simulink library "Multibody_Parts_Lib"  (R2024a)
settings: Solver=VariableStepAuto  StartTime=0.0  StopTime=10.0  RelTol=1e-3
undefined symbols (not defined in the file or in its folder): b_gear_pd_asy, b_radius_asy, b_visc_frict_asy, bevel_angle_asy, bevel_angle_bf_asy, bevel_angle_fg_asy, f_gear_pd_asy, f_radius_asy, f_visc_frict_asy, g_radius_asy, g_visc_frict_asy, gear_ra_asy, gear_visc_frict_asy, Hand, Left, Local, pinion_pd_asy, screw_lead, worm_lead_angle_asy, worm_rad_asy, worm_visc_frict_asy, X, Y, Z
libraries: sm_lib x143, $bdroot x22, nesl_utility x16
(part 6 of 6)

== system Multibody_Parts_Lib/Gears/Assemblies/Bevel Gear Assembly ==
  Constraints : $bdroot/Gears/Assemblies/Bevel Gear Constraints  bevel_angle=bevel_angle_asy  b_radius=b_radius_asy  f_radius=f_radius_asy  b_visc_frict=b_visc_frict_asy  f_visc_frict=f_visc_frict_asy
  Gear B : $bdroot/Gears/Bevel Gear  gear_ra=b_radius_asy  gear_th=b_thickness_asy  gear_ca=b_cone_angle_asy  gear_hr=b_hole_radius_asy  gear_rho=b_rho_asy  gear_clr=b_clr_asy  gear_opc=b_opc_asy  popup_markings=Two  mark_radius_range=b_mark_radius_range  mark_angle_range=b_mark_angle_range  mark_color=b_mark_clr
  Gear F : $bdroot/Gears/Bevel Gear  gear_ra=f_radius_asy  gear_th=f_thickness_asy  gear_ca=bevel_angle_asy-b_cone_angle_asy  gear_hr=f_hole_radius_asy  gear_rho=f_rho_asy  gear_clr=f_clr_asy  gear_opc=f_opc_asy  popup_markings=Two  mark_radius_range=f_mark_radius_range  mark_angle_range=f_mark_angle_range  mark_color=f_mark_clr
  F : PMIOPort  Side=Left
  B : PMIOPort  Port=2  Side=Left
  H : PMIOPort  Port=3  Side=Left
  connections:
  Constraints/LConn2 -- Gear B/RConn1 -- B/RConn1
  Constraints/LConn1 -- Gear F/RConn1 -- F/RConn1
  Constraints/LConn3 -- H/RConn1

== system Multibody_Parts_Lib/Gears/Assemblies/Common Gear Constraints ==
  Common Gear Constraint : sm_lib/Gears and Couplings/Gears/Common Gear Constraint  GearType=External  SpecificationType=PitchCircleRadii  CenterDistance=30  CenterDistanceUnits=cm  GearRatio=0.5  BaseGearRadius=b_gear_pd/2  BaseGearRadiusUnits=m  FollGearRadius=f_gear_pd/2  FollGearRadiusUnits=m
  Revolute Gear B : sm_lib/Joints/Revolute Joint  JointMode=Normal  CompositeWrenchDir=FollowerOnBase  CompositeWrenchFrame=BaseFrame  SenseConstraintForce=off  SenseConstraintTorque=off  SenseTotalForce=off  SenseTotalTorque=off  PositionTargetSpecify=off  PositionTargetPriority=High  PositionTargetValue=0  PositionTargetValueUnits=deg  VelocityTargetSpecify=off  VelocityTargetPriority=High  VelocityTargetValue=0  VelocityTargetValueUnits=deg/s  EquilibriumPosition=0  EquilibriumPositionUnits=deg  SpringStiffness=0  SpringStiffnessUnits=N*m/deg  DampingCoefficient=b_visc_frict  DampingCoefficientUnits=N*m/(deg/s)  LowerLimitSpecify=off  LowerLimitBound=-90  LowerLimitBoundUnits=deg  LowerLimitStiffness=1e4  LowerLimitStiffnessUnits=N*m/deg  LowerLimitDamping=10  LowerLimitDampingUnits=N*m/(deg/s)  LowerLimitTransitionRegionWidth=0.1  LowerLimitTransitionRegionWidthUnits=deg  UpperLimitSpecify=off  UpperLimitBound=90  UpperLimitBoundUnits=deg  UpperLimitStiffness=1e4  UpperLimitStiffnessUnits=N*m/deg  UpperLimitDamping=10  UpperLimitDampingUnits=N*m/(deg/s)  UpperLimitTransitionRegionWidth=0.1  UpperLimitTransitionRegionWidthUnits=deg  TorqueActuationMode=NoTorque  MotionActuationMode=ComputedMotion  SensePosition=off  SenseVelocity=off  SenseAcceleration=off  SenseTorqueForce=off  SenseLowerLimitTorqueForce=off  SenseUpperLimitTorqueForce=off
  Revolute Gear F : sm_lib/Joints/Revolute Joint  JointMode=Normal  CompositeWrenchDir=FollowerOnBase  CompositeWrenchFrame=BaseFrame  SenseConstraintForce=off  SenseConstraintTorque=off  SenseTotalForce=off  SenseTotalTorque=off  PositionTargetSpecify=on  PositionTargetPriority=High  PositionTargetValue=45  PositionTargetValueUnits=deg  VelocityTargetSpecify=off  VelocityTargetPriority=High  VelocityTargetValue=0  VelocityTargetValueUnits=deg/s  EquilibriumPosition=0  EquilibriumPositionUnits=deg  SpringStiffness=0  SpringStiffnessUnits=N*m/deg  DampingCoefficient=f_visc_frict  DampingCoefficientUnits=N*m/(deg/s)  LowerLimitSpecify=off  LowerLimitBound=-90  LowerLimitBoundUnits=deg  LowerLimitStiffness=1e4  LowerLimitStiffnessUnits=N*m/deg  LowerLimitDamping=10  LowerLimitDampingUnits=N*m/(deg/s)  LowerLimitTransitionRegionWidth=0.1  LowerLimitTransitionRegionWidthUnits=deg  UpperLimitSpecify=off  UpperLimitBound=90  UpperLimitBoundUnits=deg  UpperLimitStiffness=1e4  UpperLimitStiffnessUnits=N*m/deg  UpperLimitDamping=10  UpperLimitDampingUnits=N*m/(deg/s)  UpperLimitTransitionRegionWidth=0.1  UpperLimitTransitionRegionWidthUnits=deg  TorqueActuationMode=NoTorque  MotionActuationMode=ComputedMotion  SensePosition=off  SenseVelocity=off  SenseAcceleration=off  SenseTorqueForce=off  SenseLowerLimitTorqueForce=off  SenseUpperLimitTorqueForce=off
  Transform Gear F : sm_lib/Frames and Transforms/Rigid Transform  RotationMethod=None  FollAlignAxisA=+X  BaseAlignAxisA=+Y  FollAlignAxisB=+Y  BaseAlignAxisB=+Z  RotationStandardAxis=+Z  RotationAngle=0  RotationAngleUnits=deg  RotationArbitraryAxis=[0 0 1]  RotationSequenceAxes=FollowerAxes  RotationSequence=XYX  RotationSequenceAngles=[0 0 0]  RotationSequenceAnglesUnits=deg  RotationMatrix=[1 0 0; 0 1 0; 0 0 1]  Quaternion=[1 0 0 0]  TranslationMethod=StandardAxis  TranslationCartesianOffset=[0 0 0]  TranslationCartesianOffsetUnits=m  TranslationStandardAxis=+X  TranslationStandardOffset=gear_axis_offset  TranslationStandardOffsetUnits=m  TranslationROffset=0  TranslationROffsetUnits=m  TranslationThetaOffset=0  TranslationThetaOffsetUnits=deg  TranslationZOffset=0  TranslationZOffsetUnits=m
  F : PMIOPort  Side=Left
  B : PMIOPort  Port=2  Side=Left
  H : PMIOPort  Port=3  Side=Left
  connections:
  Revolute Gear B/RConn1 -- Common Gear Constraint/LConn1 -- B/RConn1
  Revolute Gear F/RConn1 -- Common Gear Constraint/RConn1 -- F/RConn1
  Transform Gear F/RConn1 -- Revolute Gear F/LConn1
  H/RConn1 -- Transform Gear F/LConn1 -- Revolute Gear B/LConn1

== system Multibody_Parts_Lib/Gears/Assemblies/Common Gear Assembly ==
  Constraints : $bdroot/Gears/Assemblies/Common Gear Constraints  popup_gear_type=External  b_gear_pd=b_gear_pd_asy  f_gear_pd=f_gear_pd_asy  b_visc_frict=b_visc_frict_asy  f_visc_frict=f_visc_frict_asy
  Gear B : $bdroot/Gears/Gear  popup_gear_type=External  gear_pd=b_gear_pd_asy  gear_nt=b_gear_nt  gear_th=b_gear_th  gear_rh=b_gear_rh  gear_rt=pinion_rt  gear_rho=b_gear_rho  gear_clr=b_gear_clr  gear_opc=b_gear_opc  popup_ad_dd=Specify  gear_ad=b_gear_ad  gear_dd=b_gear_dd  popup_markings=Two  mark_radius_range=b_mark_radius_range  mark_angle_range=b_mark_angle_range  mark_color=b_mark_color
  Gear F : $bdroot/Gears/Gear  popup_gear_type=External  gear_pd=f_gear_pd_asy  gear_nt=f_gear_nt  gear_th=f_gear_th  gear_rh=f_gear_rht  gear_rt=f_gear_rht  gear_rho=f_gear_rho  gear_clr=f_gear_clr  gear_opc=f_gear_opc  popup_ad_dd=Specify  gear_ad=f_gear_ad  gear_dd=f_gear_dd  popup_markings=Two  mark_radius_range=f_mark_radius_range  mark_angle_range=f_mark_angle_range  mark_color=f_mark_color
  Transform B Offset Angle : sm_lib/Frames and Transforms/Rigid Transform  RotationMethod=StandardAxis  FollAlignAxisA=+X  BaseAlignAxisA=+Y  FollAlignAxisB=+Y  BaseAlignAxisB=+Z  RotationStandardAxis=+Z  RotationAngle=b_gear_offset_angle  RotationAngleUnits=deg  RotationArbitraryAxis=[0 0 1]  RotationSequenceAxes=FollowerAxes  RotationSequence=XYX  RotationSequenceAngles=[0 0 0]  RotationSequenceAnglesUnits=deg  RotationMatrix=[1 0 0; 0 1 0; 0 0 1]  Quaternion=[1 0 0 0]  TranslationMethod=None  TranslationCartesianOffset=[0 0 0]  TranslationCartesianOffsetUnits=m  TranslationStandardAxis=+Z  TranslationStandardOffset=0  TranslationStandardOffsetUnits=m  TranslationROffset=0  TranslationROffsetUnits=m  TranslationThetaOffset=0  TranslationThetaOffsetUnits=deg  TranslationZOffset=0  TranslationZOffsetUnits=m
  Transform F Offset Angle : sm_lib/Frames and Transforms/Rigid Transform  RotationMethod=StandardAxis  FollAlignAxisA=+X  BaseAlignAxisA=+Y  FollAlignAxisB=+Y  BaseAlignAxisB=+Z  RotationStandardAxis=+Z  RotationAngle=f_gear_offset_angle  RotationAngleUnits=deg  RotationArbitraryAxis=[0 0 1]  RotationSequenceAxes=FollowerAxes  RotationSequence=XYX  RotationSequenceAngles=[0 0 0]  RotationSequenceAnglesUnits=deg  RotationMatrix=[1 0 0; 0 1 0; 0 0 1]  Quaternion=[1 0 0 0]  TranslationMethod=None  TranslationCartesianOffset=[0 0 0]  TranslationCartesianOffsetUnits=m  TranslationStandardAxis=+Z  TranslationStandardOffset=0  TranslationStandardOffsetUnits=m  TranslationROffset=0  TranslationROffsetUnits=m  TranslationThetaOffset=0  TranslationThetaOffsetUnits=deg  TranslationZOffset=0  TranslationZOffsetUnits=m
  F : PMIOPort  Side=Left
  B : PMIOPort  Port=2  Side=Left
  H : PMIOPort  Port=3  Side=Left
  connections:
  Constraints/LConn3 -- H/RConn1
  Gear B/RConn1 -- Transform B Offset Angle/RConn1
  Gear F/RConn1 -- Transform F Offset Angle/RConn1
  F/RConn1 -- Constraints/LConn1 -- Transform F Offset Angle/LConn1
  Constraints/LConn2 -- B/RConn1 -- Transform B Offset Angle/LConn1

== system Multibody_Parts_Lib/Gears/Assemblies/Rack and Pinion Constraints ==
  Check Frames Rack and Pinion : Subsystem
  Prismatic Rack : sm_lib/Joints/Prismatic Joint  JointMode=Normal  CompositeWrenchDir=FollowerOnBase  CompositeWrenchFrame=BaseFrame  SenseConstraintForce=off  SenseConstraintTorque=off  SenseTotalForce=off  SenseTotalTorque=off  PositionTargetSpecify=off  PositionTargetPriority=High  PositionTargetValue=0  PositionTargetValueUnits=m  VelocityTargetSpecify=off  VelocityTargetPriority=High  VelocityTargetValue=0  VelocityTargetValueUnits=m/s  EquilibriumPosition=0  EquilibriumPositionUnits=m  SpringStiffness=0  SpringStiffnessUnits=N/m  DampingCoefficient=rack_visc_frict  DampingCoefficientUnits=N/(m/s)  LowerLimitSpecify=off  LowerLimitBound=-1  LowerLimitBoundUnits=m  LowerLimitStiffness=1e6  LowerLimitStiffnessUnits=N/m  LowerLimitDamping=1e3  LowerLimitDampingUnits=N/(m/s)  LowerLimitTransitionRegionWidth=1e-4  LowerLimitTransitionRegionWidthUnits=m  UpperLimitSpecify=off  UpperLimitBound=1  UpperLimitBoundUnits=m  UpperLimitStiffness=1e6  UpperLimitStiffnessUnits=N/m  UpperLimitDamping=1e3  UpperLimitDampingUnits=N/(m/s)  UpperLimitTransitionRegionWidth=1e-4  UpperLimitTransitionRegionWidthUnits=m  TorqueActuationMode=NoTorque  MotionActuationMode=ComputedMotion  SensePosition=off  SenseVelocity=off  SenseAcceleration=off  SenseTorqueForce=off  SenseLowerLimitTorqueForce=off  SenseUpperLimitTorqueForce=off
  Rack and Pinion Constraint : sm_lib/Gears and Couplings/Gears/Rack and Pinion Constraint  PinionRadius=pinion_pd/2  PinionRadiusUnits=m
  Revolute Pinion : sm_lib/Joints/Revolute Joint  JointMode=Normal  CompositeWrenchDir=FollowerOnBase  CompositeWrenchFrame=BaseFrame  SenseConstraintForce=off  SenseConstraintTorque=off  SenseTotalForce=off  SenseTotalTorque=off  PositionTargetSpecify=off  PositionTargetPriority=High  PositionTargetValue=15  PositionTargetValueUnits=deg  VelocityTargetSpecify=off  VelocityTargetPriority=High  VelocityTargetValue=0  VelocityTargetValueUnits=deg/s  EquilibriumPosition=0  EquilibriumPositionUnits=deg  SpringStiffness=0  SpringStiffnessUnits=N*m/deg  DampingCoefficient=pinion_visc_frict  DampingCoefficientUnits=N*m/(deg/s)  LowerLimitSpecify=off  LowerLimitBound=-90  LowerLimitBoundUnits=deg  LowerLimitStiffness=1e4  LowerLimitStiffnessUnits=N*m/deg  LowerLimitDamping=10  LowerLimitDampingUnits=N*m/(deg/s)  LowerLimitTransitionRegionWidth=0.1  LowerLimitTransitionRegionWidthUnits=deg  UpperLimitSpecify=off  UpperLimitBound=90  UpperLimitBoundUnits=deg  UpperLimitStiffness=1e4  UpperLimitStiffnessUnits=N*m/deg  UpperLimitDamping=10  UpperLimitDampingUnits=N*m/(deg/s)  UpperLimitTransitionRegionWidth=0.1  UpperLimitTransitionRegionWidthUnits=deg  TorqueActuationMode=NoTorque  MotionActuationMode=ComputedMotion  SensePosition=off  SenseVelocity=off  SenseAcceleration=off  SenseTorqueForce=off  SenseLowerLimitTorqueForce=off  SenseUpperLimitTorqueForce=off
  Transform Pinion : sm_lib/Frames and Transforms/Rigid Transform  RotationMethod=StandardAxis  FollAlignAxisA=+X  BaseAlignAxisA=+Y  FollAlignAxisB=+Y  BaseAlignAxisB=+Z  RotationStandardAxis=+Y  RotationAngle=-90  RotationAngleUnits=deg  RotationArbitraryAxis=[0 0 1]  RotationSequenceAxes=FollowerAxes  RotationSequence=XYX  RotationSequenceAngles=[0 0 0]  RotationSequenceAnglesUnits=deg  RotationMatrix=[1 0 0; 0 1 0; 0 0 1]  Quaternion=[1 0 0 0]  TranslationMethod=StandardAxis  TranslationCartesianOffset=[0 0 0]  TranslationCartesianOffsetUnits=m  TranslationStandardAxis=+Y  TranslationStandardOffset=pinion_pd/2  TranslationStandardOffsetUnits=m  TranslationROffset=0  TranslationROffsetUnits=m  TranslationThetaOffset=0  TranslationThetaOffsetUnits=deg  TranslationZOffset=0  TranslationZOffsetUnits=m
  P : PMIOPort  Side=Left
  R : PMIOPort  Port=2  Side=Left
  H : PMIOPort  Port=3  Side=Left
  connections:
  Rack and Pinion Constraint/RConn1 -- R/RConn1 -- Prismatic Rack/RConn1 -- Check Frames Rack and Pinion/RConn2
  Revolute Pinion/LConn1 -- Transform Pinion/RConn1
  H/RConn1 -- Prismatic Rack/LConn1 -- Transform Pinion/LConn1
  P/RConn1 -- Revolute Pinion/RConn1 -- Rack and Pinion Constraint/LConn1 -- Check Frames Rack and Pinion/RConn1

== system Multibody_Parts_Lib/Gears/Assemblies/Rack and Pinion Assembly ==
  Constraints : $bdroot/Gears/Assemblies/Rack and Pinion Constraints  pinion_pd=pinion_pd_asy  pinion_visc_frict=pinion_visc_frict_asy  rack_visc_frict=rack_visc_frict_asy
  Pinion : $bdroot/Gears/Gear  popup_gear_type=External  gear_pd=pinion_pd_asy  gear_nt=pinion_nt_asy  gear_th=pinion_th_asy  gear_rh=pinion_rh_asy  gear_rt=pinion_rt  gear_rho=pinion_rho_asy  gear_clr=pinion_clr_asy  gear_opc=pinion_opc_asy  popup_ad_dd=Default  gear_ad=pinion_ad_asy  gear_dd=pinion_dd_asy  popup_markings=Two  mark_radius_range=p_mark_radius_range  mark_angle_range=p_mark_angle_range  mark_color=p_mark_color
  Rack : $bdroot/Gears/Rack  rack_tp=rack_tp_asy  rack_nt=rack_nt_asy  rack_tb=rack_tb_asy  rack_th=rack_th_asy  rack_rho=rack_rho_asy  rack_clr=rack_clr_asy  rack_opc=rack_opc_asy  popup_ad_dd=Default  rack_ad=rack_ad_asy  rack_dd=rack_dd_asy
  P : PMIOPort  Side=Left
  R : PMIOPort  Port=2  Side=Left
  H : PMIOPort  Port=3  Side=Left
  connections:
  Constraints/LConn3 -- H/RConn1
  Constraints/LConn2 -- Rack/RConn1 -- R/RConn1
  Constraints/LConn1 -- Pinion/RConn1 -- P/RConn1

== system Multibody_Parts_Lib/Gears/Assemblies/Worm Gear Constraints ==
  Revolute Gear : sm_lib/Joints/Revolute Joint  JointMode=Normal  CompositeWrenchDir=FollowerOnBase  CompositeWrenchFrame=BaseFrame  SenseConstraintForce=off  SenseConstraintTorque=off  SenseTotalForce=off  SenseTotalTorque=off  PositionTargetSpecify=off  PositionTargetPriority=High  PositionTargetValue=0  PositionTargetValueUnits=deg  VelocityTargetSpecify=off  VelocityTargetPriority=High  VelocityTargetValue=0  VelocityTargetValueUnits=deg/s  EquilibriumPosition=0  EquilibriumPositionUnits=deg  SpringStiffness=0  SpringStiffnessUnits=N*m/deg  DampingCoefficient=gear_visc_frict  DampingCoefficientUnits=N*m/(deg/s)  LowerLimitSpecify=off  LowerLimitBound=-90  LowerLimitBoundUnits=deg  LowerLimitStiffness=1e4  LowerLimitStiffnessUnits=N*m/deg  LowerLimitDamping=10  LowerLimitDampingUnits=N*m/(deg/s)  LowerLimitTransitionRegionWidth=0.1  LowerLimitTransitionRegionWidthUnits=deg  UpperLimitSpecify=off  UpperLimitBound=90  UpperLimitBoundUnits=deg  UpperLimitStiffness=1e4  UpperLimitStiffnessUnits=N*m/deg  UpperLimitDamping=10  UpperLimitDampingUnits=N*m/(deg/s)  UpperLimitTransitionRegionWidth=0.1  UpperLimitTransitionRegionWidthUnits=deg  TorqueActuationMode=NoTorque  MotionActuationMode=ComputedMotion  SensePosition=off  SenseVelocity=off  SenseAcceleration=off  SenseTorqueForce=off  SenseLowerLimitTorqueForce=off  SenseUpperLimitTorqueForce=off
  Revolute Worm : sm_lib/Joints/Revolute Joint  JointMode=Normal  CompositeWrenchDir=FollowerOnBase  CompositeWrenchFrame=BaseFrame  SenseConstraintForce=off  SenseConstraintTorque=off  SenseTotalForce=off  SenseTotalTorque=off  PositionTargetSpecify=off  PositionTargetPriority=High  PositionTargetValue=0  PositionTargetValueUnits=deg  VelocityTargetSpecify=off  VelocityTargetPriority=High  VelocityTargetValue=0  VelocityTargetValueUnits=deg/s  EquilibriumPosition=0  EquilibriumPositionUnits=deg  SpringStiffness=0  SpringStiffnessUnits=N*m/deg  DampingCoefficient=worm_visc_frict  DampingCoefficientUnits=N*m/(deg/s)  LowerLimitSpecify=off  LowerLimitBound=-90  LowerLimitBoundUnits=deg  LowerLimitStiffness=1e4  LowerLimitStiffnessUnits=N*m/deg  LowerLimitDamping=10  LowerLimitDampingUnits=N*m/(deg/s)  LowerLimitTransitionRegionWidth=0.1  LowerLimitTransitionRegionWidthUnits=deg  UpperLimitSpecify=off  UpperLimitBound=90  UpperLimitBoundUnits=deg  UpperLimitStiffness=1e4  UpperLimitStiffnessUnits=N*m/deg  UpperLimitDamping=10  UpperLimitDampingUnits=N*m/(deg/s)  UpperLimitTransitionRegionWidth=0.1  UpperLimitTransitionRegionWidthUnits=deg  TorqueActuationMode=NoTorque  MotionActuationMode=ComputedMotion  SensePosition=off  SenseVelocity=off  SenseAcceleration=off  SenseTorqueForce=off  SenseLowerLimitTorqueForce=off  SenseUpperLimitTorqueForce=off
  Transform Gear : sm_lib/Frames and Transforms/Rigid Transform  RotationMethod=StandardAxis  FollAlignAxisA=+X  BaseAlignAxisA=+Y  FollAlignAxisB=+Y  BaseAlignAxisB=+Z  RotationStandardAxis=+Y  RotationAngle=90  RotationAngleUnits=deg  RotationArbitraryAxis=[0 0 1]  RotationSequenceAxes=FollowerAxes  RotationSequence=XYX  RotationSequenceAngles=[0 0 0]  RotationSequenceAnglesUnits=deg  RotationMatrix=[1 0 0; 0 1 0; 0 0 1]  Quaternion=[1 0 0 0]  TranslationMethod=StandardAxis  TranslationCartesianOffset=[0 0 0]  TranslationCartesianOffsetUnits=m  TranslationStandardAxis=+Y  TranslationStandardOffset=worm_rad+gear_rad  TranslationStandardOffsetUnits=m  TranslationROffset=0  TranslationROffsetUnits=m  TranslationThetaOffset=0  TranslationThetaOffsetUnits=deg  TranslationZOffset=0  TranslationZOffsetUnits=m
  Worm and Gear Constraint : sm_lib/Gears and Couplings/Gears/Worm and Gear Constraint  WormDirection=LeftHand  WormLeadAngle=worm_lead_angle  WormLeadAngleUnits=deg  SpecificationMethod=PitchCircleRadii  CenterDistance=20  CenterDistanceUnits=cm  Ratio=1  WormRadius=worm_rad  WormRadiusUnits=m  GearRadius=gear_rad  GearRadiusUnits=m
  G : PMIOPort  Side=Left
  W : PMIOPort  Port=2  Side=Left
  H : PMIOPort  Port=3  Side=Left
  connections:
  W/RConn1 -- Revolute Worm/RConn1 -- Worm and Gear Constraint/LConn1
  H/RConn1 -- Transform Gear/LConn1 -- Revolute Worm/LConn1
  Revolute Gear/LConn1 -- Transform Gear/RConn1
  G/RConn1 -- Revolute Gear/RConn1 -- Worm and Gear Constraint/RConn1

== system Multibody_Parts_Lib/Gears/Assemblies/Worm Gear Assembly ==
  Constraints : $bdroot/Gears/Assemblies/Worm Gear Constraints  popup_worm_dir=Left-Hand  worm_lead_angle=worm_lead_angle_asy  worm_rad=worm_rad_asy  gear_rad=gear_ra_asy  worm_visc_frict=worm_visc_frict_asy  gear_visc_frict=gear_visc_frict_asy
  Gear : $bdroot/Basic/Cylinder  cyl_ra=37.5e-3  cyl_th=9e-3  cyl_hr=5e-3  cyl_rho=7000  cyl_clr=[0.6 0.6 0.6]  cyl_opc=1  popup_markings=Two  mark_radius_range=g_mark_radius_range  mark_angle_range=g_mark_angle_range  mark_color=g_mark_color
  WormB : $bdroot/Basic/Rod  rod_rad=worm_rad_asy  rod_len=worm_len_asy/2  rod_rho=worm_rho_asy  rod_color=worm_color_asy  rod_opc=1  popup_zori=Local +Z  popup_markings=Two  mark_radius_range=w_mark_radius_range  mark_length_range=w_mark_length_range  mark_angle_range=w_mark_angle_range  mark_color=w_mark_color
  WormF : $bdroot/Basic/Rod  rod_rad=worm_rad_asy  rod_len=worm_len_asy/2  rod_rho=worm_rho_asy  rod_color=worm_color_asy  rod_opc=1  popup_zori=Local +Z  popup_markings=Two  mark_radius_range=w_mark_radius_range  mark_length_range=w_mark_length_range  mark_angle_range=w_mark_angle_range  mark_color=w_mark_color
  G : PMIOPort  Side=Left
  W : PMIOPort  Port=2  Side=Left
  H : PMIOPort  Port=3  Side=Left
  connections:
  Constraints/LConn3 -- H/RConn1
  Constraints/LConn1 -- Gear/RConn1 -- G/RConn1
  WormB/RConn1 -- Constraints/LConn2 -- W/RConn1 -- WormF/LConn1

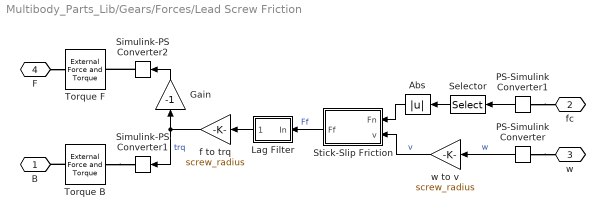
== system Multibody_Parts_Lib/Gears/Forces/Lead Screw Friction ==
  Abs : Abs  SaturateOnIntegerOverflow=off
  Gain : Gain  Gain=-1
  Lag Filter : Subsystem  mask(First-order lag supporting vector signals){b=filt_const, x_initial=0}
      mask prompts: b "Filter time constant"; x_initial "Initial output"
      mask help: Models a lag of the form 1/(b*s+1) where s is the Laplace operator.
  PS-Simulink Converter : nesl_utility/PS-Simulink Converter  PhysicalDomain=network_engine_domain  SubClassName=ps_output  LeftPortType=input  RightPortType=output  PseudoPeriodic=off  Frequencies=[]  VectorFormat=1-D array  Unit=1  AffineConversion=off
  PS-Simulink Converter1 : nesl_utility/PS-Simulink Converter  PhysicalDomain=network_engine_domain  SubClassName=ps_output  LeftPortType=input  RightPortType=output  PseudoPeriodic=off  Frequencies=[]  VectorFormat=1-D array  Unit=1  AffineConversion=off
  Selector : Selector  InputPortWidth=3  IndexOptions=Index vector (dialog)  Indices=[3]  OutputSizes=1
  Simulink-PS Converter1 : nesl_utility/Simulink-PS Converter  PhysicalDomain=network_engine_domain  SubClassName=ps_input  LeftPortType=input  RightPortType=output  PseudoPeriodic=off  Frequencies=[]  NoiseDistribution=none  NoiseParameters=[]  Unit=1  AffineConversion=off  FilteringAndDerivatives=zero  SimscapeFilterOrder=2  InputFilterTimeConstant=0.01  UdotUserProvided=1
  Simulink-PS Converter2 : nesl_utility/Simulink-PS Converter  PhysicalDomain=network_engine_domain  SubClassName=ps_input  LeftPortType=input  RightPortType=output  PseudoPeriodic=off  Frequencies=[]  NoiseDistribution=none  NoiseParameters=[]  Unit=1  AffineConversion=off  FilteringAndDerivatives=zero  SimscapeFilterOrder=2  InputFilterTimeConstant=0.01  UdotUserProvided=1
  "Stick-Slip Friction " : Subsystem  VariantControl=Stick_Slip_C  mask(Stick-Slip Friction, Continuous){muk=mu_kinetic, mus=mu_static, vth=vel_th}
      mask prompts: muk "Coefficient of Kinetic Friction"; mus "Coefficient of Static Friction"; vth "Velocity Threshold (m/s)"
      mask help: Implements a continuous stick-slip friction model. Smaller velocity threshold is closer to reality but results in a numerically stiffer system.
  Torque B : sm_lib/Forces and Torques/External Force and Torque  EnableForceX=off  EnableForceY=off  EnableForceZ=off  EnableForce=off  ForceResolutionFrame=AttachedFrame  EnableTorqueX=off  EnableTorqueY=off  EnableTorqueZ=on  EnableTorque=off  TorqueResolutionFrame=AttachedFrame
  Torque F : sm_lib/Forces and Torques/External Force and Torque  EnableForceX=off  EnableForceY=off  EnableForceZ=off  EnableForce=off  ForceResolutionFrame=AttachedFrame  EnableTorqueX=off  EnableTorqueY=off  EnableTorqueZ=on  EnableTorque=off  TorqueResolutionFrame=AttachedFrame
  f to trq : Gain  Gain=screw_radius
      settings: AttributesFormatString=%<Gain>
  w to v : Gain  Gain=screw_radius
      settings: AttributesFormatString=%<Gain>
  B : PMIOPort  Side=Right
  fc : PMIOPort  Port=2  Side=Left
  w : PMIOPort  Port=3  Side=Left
  F : PMIOPort  Port=4  Side=Left
  wires:
  Lag Filter/1(Out) -> f to trq/1
  Selector/1 -> Abs/1
  Gain/1 -> Simulink-PS Converter2/1
  w to v/1 -> "Stick-Slip Friction "/2(v)  "v"
  f to trq/1 -> Simulink-PS Converter1/1, Gain/1  "trq"
  Abs/1 -> "Stick-Slip Friction "/1(Fn)
  PS-Simulink Converter1/1 -> Selector/1
  PS-Simulink Converter/1 -> w to v/1  "w"
  "Stick-Slip Friction "/1(Ff) -> Lag Filter/1(In)  "Ff"
  connections:
  F/RConn1 -- Torque F/RConn1
  Simulink-PS Converter2/RConn1 -- Torque F/LConn1
  Torque B/RConn1 -- B/RConn1
  Torque B/LConn1 -- Simulink-PS Converter1/RConn1
  PS-Simulink Converter/LConn1 -- w/RConn1
  PS-Simulink Converter1/LConn1 -- fc/RConn1

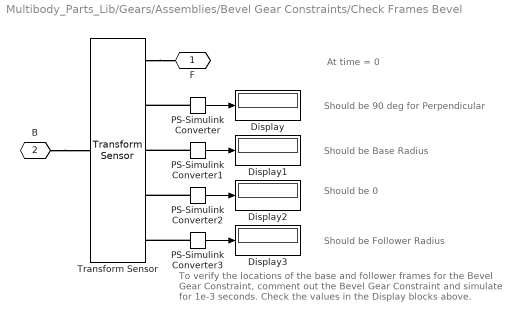
== system Multibody_Parts_Lib/Gears/Assemblies/Bevel Gear Constraints/Check Frames Bevel ==
  note: To verify the locations of the base and follower frames for the Bevel Gear Constraint, comment out the Bevel Gear Constraint and simulate for 1e-3 seconds. Check the values in the Display blocks above.
  note: Should be Follower Radius
  note: Should be 0
  note: Should be 90 deg for Perpendicular
  note: Should be Base Radius
  note: At time = 0
  Display{,1..3} (4 alike) : Display
      settings: Decimation=1e5
  PS-Simulink Converter : nesl_utility/PS-Simulink Converter  PhysicalDomain=network_engine_domain  SubClassName=ps_output  LeftPortType=input  RightPortType=output  PseudoPeriodic=off  Frequencies=[]  VectorFormat=1-D array  Unit=deg  AffineConversion=off
  PS-Simulink Converter1 : nesl_utility/PS-Simulink Converter  PhysicalDomain=network_engine_domain  SubClassName=ps_output  LeftPortType=input  RightPortType=output  PseudoPeriodic=off  Frequencies=[]  VectorFormat=1-D array  Unit=1  AffineConversion=off
  PS-Simulink Converter2 : nesl_utility/PS-Simulink Converter  PhysicalDomain=network_engine_domain  SubClassName=ps_output  LeftPortType=input  RightPortType=output  PseudoPeriodic=off  Frequencies=[]  VectorFormat=1-D array  Unit=1  AffineConversion=off
  PS-Simulink Converter3 : nesl_utility/PS-Simulink Converter  PhysicalDomain=network_engine_domain  SubClassName=ps_output  LeftPortType=input  RightPortType=output  PseudoPeriodic=off  Frequencies=[]  VectorFormat=1-D array  Unit=1  AffineConversion=off
  Transform Sensor : sm_lib/Frames and Transforms/Transform Sensor  MeasurementFrame=World  RotationSequence=XYX  SenseAngle=on  SenseAxis=off  SenseQ=off  SenseR=off  SenseRotationSequence=off  SenseOmegaX=off  SenseOmegaY=off  SenseOmegaZ=off  SenseOmega=off  SenseQDot=off  SenseRDot=off  SenseRotationSequenceDot=off  SenseAlphaX=off  SenseAlphaY=off  SenseAlphaZ=off  SenseAlpha=off  SenseQDDot=off  SenseRDDot=off  SenseX=on  SenseY=on  SenseZ=on  SenseXYZ=off  SenseRad=off  SenseAzim=off  SenseDist=off  SenseInc=off  SenseXDot=off  SenseYDot=off  SenseZDot=off  SenseXYZDot=off  SenseRadDot=off  SenseAzimDot=off  SenseDistDot=off  SenseIncDot=off  SenseXDDot=off  SenseYDDot=off  SenseZDDot=off  SenseXYZDDot=off  SenseRadDDot=off  SenseAzimDDot=off  SenseDistDDot=off  SenseIncDDot=off
  F : PMIOPort  Side=Right
  B : PMIOPort  Port=2  Side=Right
  wires:
  PS-Simulink Converter1/1 -> Display1/1
  PS-Simulink Converter2/1 -> Display2/1
  PS-Simulink Converter/1 -> Display/1
  PS-Simulink Converter3/1 -> Display3/1
  connections:
  PS-Simulink Converter2/LConn1 -- Transform Sensor/RConn4
  PS-Simulink Converter1/LConn1 -- Transform Sensor/RConn3
  PS-Simulink Converter/LConn1 -- Transform Sensor/RConn2
  PS-Simulink Converter3/LConn1 -- Transform Sensor/RConn5
  Transform Sensor/RConn1 -- F/RConn1
  B/RConn1 -- Transform Sensor/LConn1

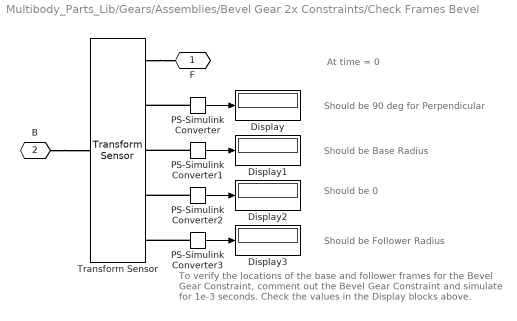
== system Multibody_Parts_Lib/Gears/Assemblies/Bevel Gear 2x Constraints/Check Frames Bevel ==
  note: To verify the locations of the base and follower frames for the Bevel Gear Constraint, comment out the Bevel Gear Constraint and simulate for 1e-3 seconds. Check the values in the Display blocks above.
  note: Should be Follower Radius
  note: Should be 0
  note: Should be 90 deg for Perpendicular
  note: Should be Base Radius
  note: At time = 0
  Display{,1..3} (4 alike) : Display
      settings: Decimation=1e5
  PS-Simulink Converter : nesl_utility/PS-Simulink Converter  PhysicalDomain=network_engine_domain  SubClassName=ps_output  LeftPortType=input  RightPortType=output  PseudoPeriodic=off  Frequencies=[]  VectorFormat=1-D array  Unit=deg  AffineConversion=off
  PS-Simulink Converter1 : nesl_utility/PS-Simulink Converter  PhysicalDomain=network_engine_domain  SubClassName=ps_output  LeftPortType=input  RightPortType=output  PseudoPeriodic=off  Frequencies=[]  VectorFormat=1-D array  Unit=1  AffineConversion=off
  PS-Simulink Converter2 : nesl_utility/PS-Simulink Converter  PhysicalDomain=network_engine_domain  SubClassName=ps_output  LeftPortType=input  RightPortType=output  PseudoPeriodic=off  Frequencies=[]  VectorFormat=1-D array  Unit=1  AffineConversion=off
  PS-Simulink Converter3 : nesl_utility/PS-Simulink Converter  PhysicalDomain=network_engine_domain  SubClassName=ps_output  LeftPortType=input  RightPortType=output  PseudoPeriodic=off  Frequencies=[]  VectorFormat=1-D array  Unit=1  AffineConversion=off
  Transform Sensor : sm_lib/Frames and Transforms/Transform Sensor  MeasurementFrame=World  RotationSequence=XYX  SenseAngle=on  SenseAxis=off  SenseQ=off  SenseR=off  SenseRotationSequence=off  SenseOmegaX=off  SenseOmegaY=off  SenseOmegaZ=off  SenseOmega=off  SenseQDot=off  SenseRDot=off  SenseRotationSequenceDot=off  SenseAlphaX=off  SenseAlphaY=off  SenseAlphaZ=off  SenseAlpha=off  SenseQDDot=off  SenseRDDot=off  SenseX=on  SenseY=on  SenseZ=on  SenseXYZ=off  SenseRad=off  SenseAzim=off  SenseDist=off  SenseInc=off  SenseXDot=off  SenseYDot=off  SenseZDot=off  SenseXYZDot=off  SenseRadDot=off  SenseAzimDot=off  SenseDistDot=off  SenseIncDot=off  SenseXDDot=off  SenseYDDot=off  SenseZDDot=off  SenseXYZDDot=off  SenseRadDDot=off  SenseAzimDDot=off  SenseDistDDot=off  SenseIncDDot=off
  F : PMIOPort  Side=Right
  B : PMIOPort  Port=2  Side=Right
  wires:
  PS-Simulink Converter1/1 -> Display1/1
  PS-Simulink Converter2/1 -> Display2/1
  PS-Simulink Converter/1 -> Display/1
  PS-Simulink Converter3/1 -> Display3/1
  connections:
  PS-Simulink Converter2/LConn1 -- Transform Sensor/RConn4
  PS-Simulink Converter1/LConn1 -- Transform Sensor/RConn3
  PS-Simulink Converter/LConn1 -- Transform Sensor/RConn2
  PS-Simulink Converter3/LConn1 -- Transform Sensor/RConn5
  Transform Sensor/RConn1 -- F/RConn1
  B/RConn1 -- Transform Sensor/LConn1

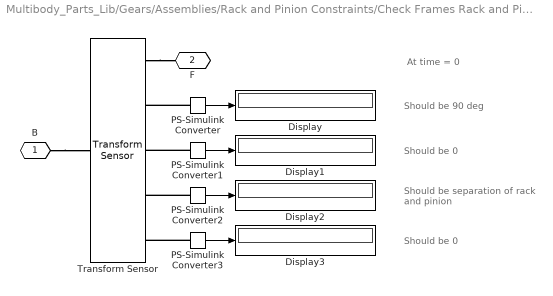
== system Multibody_Parts_Lib/Gears/Assemblies/Rack and Pinion Constraints/Check Frames Rack and Pinion ==
  note: Should be 0
  note: Should be separation
      | of rack and pinion
  note: Should be 90 deg
  note: Should be 0
  note: At time = 0
  Display{,1..3} (4 alike) : Display
      Display settings: Decimation=1e5
      Display3 settings: Decimation=1e5
  PS-Simulink Converter : nesl_utility/PS-Simulink Converter  PhysicalDomain=network_engine_domain  SubClassName=ps_output  LeftPortType=input  RightPortType=output  PseudoPeriodic=off  Frequencies=[]  VectorFormat=1-D array  Unit=deg  AffineConversion=off
  PS-Simulink Converter1 : nesl_utility/PS-Simulink Converter  PhysicalDomain=network_engine_domain  SubClassName=ps_output  LeftPortType=input  RightPortType=output  PseudoPeriodic=off  Frequencies=[]  VectorFormat=1-D array  Unit=1  AffineConversion=off
  PS-Simulink Converter2 : nesl_utility/PS-Simulink Converter  PhysicalDomain=network_engine_domain  SubClassName=ps_output  LeftPortType=input  RightPortType=output  PseudoPeriodic=off  Frequencies=[]  VectorFormat=1-D array  Unit=1  AffineConversion=off
  PS-Simulink Converter3 : nesl_utility/PS-Simulink Converter  PhysicalDomain=network_engine_domain  SubClassName=ps_output  LeftPortType=input  RightPortType=output  PseudoPeriodic=off  Frequencies=[]  VectorFormat=1-D array  Unit=1  AffineConversion=off
  Transform Sensor : sm_lib/Frames and Transforms/Transform Sensor  MeasurementFrame=World  RotationSequence=XYX  SenseAngle=on  SenseAxis=off  SenseQ=off  SenseR=off  SenseRotationSequence=off  SenseOmegaX=off  SenseOmegaY=off  SenseOmegaZ=off  SenseOmega=off  SenseQDot=off  SenseRDot=off  SenseRotationSequenceDot=off  SenseAlphaX=off  SenseAlphaY=off  SenseAlphaZ=off  SenseAlpha=off  SenseQDDot=off  SenseRDDot=off  SenseX=on  SenseY=on  SenseZ=on  SenseXYZ=off  SenseRad=off  SenseAzim=off  SenseDist=off  SenseInc=off  SenseXDot=off  SenseYDot=off  SenseZDot=off  SenseXYZDot=off  SenseRadDot=off  SenseAzimDot=off  SenseDistDot=off  SenseIncDot=off  SenseXDDot=off  SenseYDDot=off  SenseZDDot=off  SenseXYZDDot=off  SenseRadDDot=off  SenseAzimDDot=off  SenseDistDDot=off  SenseIncDDot=off
  B : PMIOPort  Side=Right
  F : PMIOPort  Port=2  Side=Right
  wires:
  PS-Simulink Converter1/1 -> Display1/1
  PS-Simulink Converter2/1 -> Display2/1
  PS-Simulink Converter/1 -> Display/1
  PS-Simulink Converter3/1 -> Display3/1
  connections:
  PS-Simulink Converter2/LConn1 -- Transform Sensor/RConn4
  PS-Simulink Converter1/LConn1 -- Transform Sensor/RConn3
  PS-Simulink Converter/LConn1 -- Transform Sensor/RConn2
  PS-Simulink Converter3/LConn1 -- Transform Sensor/RConn5
  Transform Sensor/RConn1 -- F/RConn1
  B/RConn1 -- Transform Sensor/LConn1

== system Multibody_Parts_Lib/Gears/Forces/Lead Screw Friction/Lag Filter ==
  In : Inport
  Gain : Gain  Gain=1/b
  Integrator : Integrator  InitialCondition=x_initial
  Sum : Sum  Inputs=|+-  InputSameDT=on  SaturateOnIntegerOverflow=on  OutDataTypeStr=Inherit: Same as first input
  Out : Outport  VectorParamsAs1DForOutWhenUnconnected=off
  wires:
  Gain/1 -> Out/1, Sum/2
  Integrator/1 -> Gain/1
  In/1 -> Sum/1
  Sum/1 -> Integrator/1

== system Multibody_Parts_Lib/Gears/Forces/Lead Screw Friction/Stick-Slip Friction  ==
  Fn : Inport
  v : Inport  Port=2
  Coefficient of Friction vs Velocity : Lookup_n-D  NumberOfTableDimensions=1  BreakpointsForDimension1=[-3 -1.5 -1 1 1.5 3]*vth  Table="[-muk -muk -mus mus  muk muk]"  InternalRulePriority=Speed
  Gain2 : Gain  Multiplication=Matrix(K*u)  SaturateOnIntegerOverflow=on  OutDataTypeStr=Inherit: Same as input  ParamDataTypeStr=Inherit: Same as input
  Product : Product  RndMeth=Zero
  Ff : Outport  VectorParamsAs1DForOutWhenUnconnected=off
  wires:
  Gain2/1 -> Ff/1  "Friction_Force"
  Product/1 -> Gain2/1
  v/1 -> Coefficient of Friction vs Velocity/1  "Velocity"
  Coefficient of Friction vs Velocity/1 -> Product/1
  Fn/1 -> Product/2  "Normal_Force"
